simulink model "P1"  (R2024b)
settings: Solver=VariableStepAuto  StartTime=0.0  StopTime=100  RelTol=1e-3
settings Model: Creator=sepeh  LastModifiedBy=sepeh

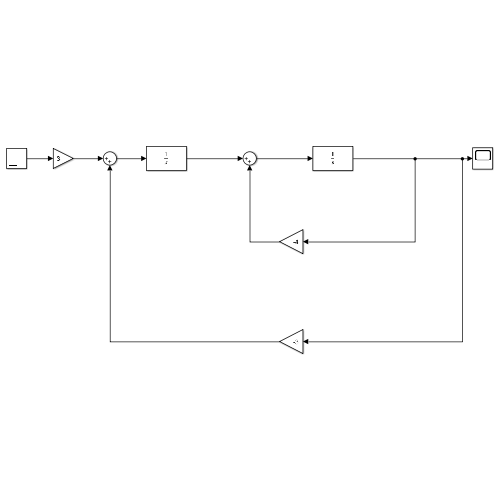
[thumbnail: Simulink's stored preview of the top-level diagram]
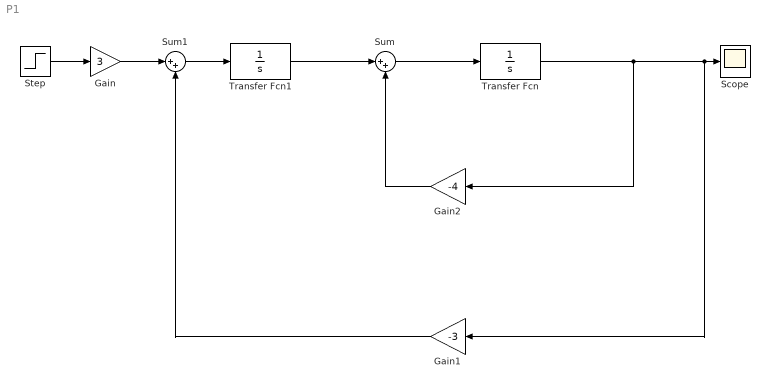
== system P1 ==
  Gain : Gain  Gain=3
  Gain1 : Gain  Gain=-3
  Gain2 : Gain  Gain=-4
  Scope : Scope
  Step : Step  SampleTime=0
  Sum : Sum  Inputs=|++
  Sum1 : Sum  Inputs=|++
  Transfer Fcn : TransferFcn  Denominator=[1 0]
  Transfer Fcn1 : TransferFcn  Denominator=[1 0]
  wires:
  Transfer Fcn1/1 -> Sum/1
  Sum/1 -> Transfer Fcn/1
  Gain/1 -> Sum1/1
  Step/1 -> Gain/1
  Sum1/1 -> Transfer Fcn1/1
  Transfer Fcn/1 -> Gain2/1, Gain1/1, Scope/1
  Gain1/1 -> Sum1/2
  Gain2/1 -> Sum/2
